simulink model "AFC1_F_trainrp_15_15_15_15_controller_ep_1000_Nor_20250519"  (R2021a)
settings: Solver=VariableStepAuto  StartTime=0.0  StopTime=10.0  RelTol=1e-3
libraries: neural x66
(part 3 of 3)

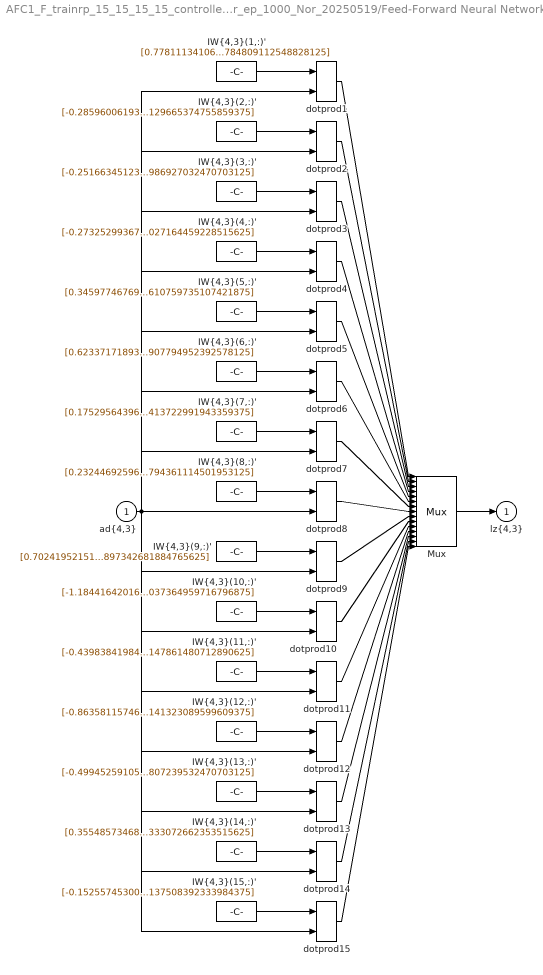
== system AFC1_F_trainrp_15_15_15_15_controller_ep_1000_Nor_20250519/Feed-Forward Neural Network/Layer 4/LW{4,3} ==
  "ad{4,3}" : Inport  PortDimensions=15
      mask Display: e = 0.06;c1 = [120 230 180]/255;c2 = ([120 230 180]+0)/(256+128);c3 = ([120 230 180]+128)/(256+128);patch([0 1 1 0],[0 0 1 1],c1);patch([0 1 1 1-e 1-e 0+e],[0 0 1 1-e 0+e 0+e],c2);patch([0 0 1 1-e 0+e 0+e],[0 1 1 1-e 1-e 0+e],c3);plot([0 1 1 0 0],[0 0 1 1 0]);
  "IW{4,3}(1,:)'" : Constant  Value=[0.7781113410617930270518627366982400417327880859375;0.62119814230305447910751581730437465012073516845703125;0.1907724978485869360422810814270633272826671600341796875;-0.29778807948838326158380596098140813410282135009765625;0.4547541881890297954527113688527606427669525146484375;-0.1544121990389732690385216073991614393889904022216796875;0.2058191613042310852410565757963922806084156036376953125;-0.404746974372004630904342548092245124280452728271484375;-0.839846360988684370596502049011178314685821533203125;0.579024458134550723542588457348756492137908935546875;1.092536353292825612726346662384457886219024658203125;0.862223254974441299935961069422774016857147216796875;0.447329224035958816774183333109249360859394073486328125;0.0023547517412946007697716055417913594283163547515869140625;0.460295474695853912283638464941759593784809112548828125]
      mask Display: e = 0.06;c1 = [120 150 230]/255;c2 = ([120 150 230]+0)/383;c3 = ([120 150 230]+128)/383;patch([0 1 1 0],[0 0 1 1],c1);patch([0 1 1 1-e 1-e 0+e],[0 0 1 1-e 0+e 0+e],c2);patch([0 0 1 1-e 0+e 0+e],[0 1 1 1-e 1-e 0+e],c3);plot([0 1 1 0 0],[0 0 1 1 0]);disp('weights');
  "IW{4,3}(10,:)'" : Constant  Value=[-1.18441642016053538810638201539404690265655517578125;0.71993919466000033668962032606941647827625274658203125;-0.73299228067737554059846161180757917463779449462890625;-1.0882850578337208702350835665129125118255615234375;-0.81389689755870031628859351258142851293087005615234375;0.80767521116610485609754732649889774620532989501953125;-0.255363153886374261158920262460014782845973968505859375;0.81081009055198982604650836947257630527019500732421875;-0.1617382409373282758924261770516750402748584747314453125;-1.1032546147443571538104833962279371917247772216796875;-0.26763008853710334999931319543975405395030975341796875;-0.5958498069031368249426350303110666573047637939453125;0.392774132323866098648323941233684308826923370361328125;-0.94132002652209190163290486452751792967319488525390625;-0.764998725995059469795478435116820037364959716796875]
      mask Display: e = 0.06;c1 = [120 150 230]/255;c2 = ([120 150 230]+0)/383;c3 = ([120 150 230]+128)/383;patch([0 1 1 0],[0 0 1 1],c1);patch([0 1 1 1-e 1-e 0+e],[0 0 1 1-e 0+e 0+e],c2);patch([0 0 1 1-e 0+e 0+e],[0 1 1 1-e 1-e 0+e],c3);plot([0 1 1 0 0],[0 0 1 1 0]);disp('weights');
  "IW{4,3}(11,:)'" : Constant  Value=[-0.43983841984739246999680517546948976814746856689453125;-0.217478877984103424747530652894056402146816253662109375;0.272952199327606448431282615274540148675441741943359375;-0.21779301126090844231697474242537282407283782958984375;-0.45534616982127251727519023916102014482021331787109375;1.2993100395773005129029797899420373141765594482421875;-0.4494260973686199367449489727732725441455841064453125;0.357711341633862922595454847396467812359333038330078125;-0.05326556157685528869460966916449251584708690643310546875;-0.72116789147178561591999823576770722866058349609375;2.368876520452326328580738845630548894405364990234375;-0.0922130686389561748939058816176839172840118408203125;-0.2799379158284567292724887010990642011165618896484375;-0.6096502573568012284255246413522399961948394775390625;0.5506923237256984293708228506147861480712890625]
      mask Display: e = 0.06;c1 = [120 150 230]/255;c2 = ([120 150 230]+0)/383;c3 = ([120 150 230]+128)/383;patch([0 1 1 0],[0 0 1 1],c1);patch([0 1 1 1-e 1-e 0+e],[0 0 1 1-e 0+e 0+e],c2);patch([0 0 1 1-e 0+e 0+e],[0 1 1 1-e 1-e 0+e],c3);plot([0 1 1 0 0],[0 0 1 1 0]);disp('weights');
  "IW{4,3}(12,:)'" : Constant  Value=[-0.86358115746454167105383703528787009418010711669921875;-0.12175056878691854767016167215842870064079761505126953125;-1.235565139600912853978798011667095124721527099609375;0.54022067020387087854516039442387409508228302001953125;0.260195066414997289161448179584112949669361114501953125;0.1290031436642831152994403964839875698089599609375;0.128307481278283452841293410529033280909061431884765625;-1.004774450547227804264593942207284271717071533203125;0.22686108419182193784990886342711746692657470703125;0.28467402097110283687442233713227324187755584716796875;4.31289008479221624980937122018076479434967041015625;-0.1441781603596583583026813357719220221042633056640625;-0.09857525629320285087686670522089116275310516357421875;0.51216925494200860047300238875322975218296051025390625;-0.24044180716196483782454151878482662141323089599609375]
      mask Display: e = 0.06;c1 = [120 150 230]/255;c2 = ([120 150 230]+0)/383;c3 = ([120 150 230]+128)/383;patch([0 1 1 0],[0 0 1 1],c1);patch([0 1 1 1-e 1-e 0+e],[0 0 1 1-e 0+e 0+e],c2);patch([0 0 1 1-e 0+e 0+e],[0 1 1 1-e 1-e 0+e],c3);plot([0 1 1 0 0],[0 0 1 1 0]);disp('weights');
  "IW{4,3}(13,:)'" : Constant  Value=[-0.49945259105140060729155493390862829983234405517578125;0.184426822089112152358580942745902575552463531494140625;-0.2031486968824770256158984693684033118188381195068359375;0.154916364295855479848995628344709984958171844482421875;0.9878538278918593817934379330836236476898193359375;0.0381209561733983626208299710924620740115642547607421875;-0.128199236742127464783180812446516938507556915283203125;0.3915529342565715609225662774406373500823974609375;0.96483039652991831047756932093761861324310302734375;0.78770085159116487449892929362249560654163360595703125;0.72610873909690687444395962302223779261112213134765625;0.93210549922399810185424939845688641071319580078125;-0.2202202028156553803572847982650273479521274566650390625;0.3195681221012935946390598473954014480113983154296875;0.7754075786498131339641304293763823807239532470703125]
      mask Display: e = 0.06;c1 = [120 150 230]/255;c2 = ([120 150 230]+0)/383;c3 = ([120 150 230]+128)/383;patch([0 1 1 0],[0 0 1 1],c1);patch([0 1 1 1-e 1-e 0+e],[0 0 1 1-e 0+e 0+e],c2);patch([0 0 1 1-e 0+e 0+e],[0 1 1 1-e 1-e 0+e],c3);plot([0 1 1 0 0],[0 0 1 1 0]);disp('weights');
  "IW{4,3}(14,:)'" : Constant  Value=[0.3554857346802153816867075875052250921726226806640625;-0.5248169129380049202637792404857464134693145751953125;0.683605962274300704706320175318978726863861083984375;-0.38434582116407411955805173420230858027935028076171875;0.58802983983653034361083200565190054476261138916015625;-0.646484905904349371752459774143062531948089599609375;0.4873657136989908433832852097111754119396209716796875;-0.1649823515269743523514733851698110811412334442138671875;0.356497028654995773422342608682811260223388671875;0.8647425210295389685910549815162084996700286865234375;0.53845365213304197116173099857405759394168853759765625;0.240110108266947452904105375637300312519073486328125;0.54410928450107098885979439728544093668460845947265625;0.53165142303777546128884523568558506667613983154296875;0.11257004837542540498507293023067177273333072662353515625]
      mask Display: e = 0.06;c1 = [120 150 230]/255;c2 = ([120 150 230]+0)/383;c3 = ([120 150 230]+128)/383;patch([0 1 1 0],[0 0 1 1],c1);patch([0 1 1 1-e 1-e 0+e],[0 0 1 1-e 0+e 0+e],c2);patch([0 0 1 1-e 0+e 0+e],[0 1 1 1-e 1-e 0+e],c3);plot([0 1 1 0 0],[0 0 1 1 0]);disp('weights');
  "IW{4,3}(15,:)'" : Constant  Value=[-0.15255745300140655107412612778716720640659332275390625;0.192276935283892225214685822720639407634735107421875;0.365743272093718096993342214773292653262615203857421875;0.6642693326831243805230542420758865773677825927734375;-0.215703456330019249787000035212258808314800262451171875;0.51382696907147706877339032871532253921031951904296875;0.398357784627120292686441871410352177917957305908203125;-0.309159641667459961222874653685721568763256072998046875;-0.650752509275324797499706619419157505035400390625;-0.454387145055632990509053570349351502954959869384765625;0.702470078125212893382922629825770854949951171875;0.3907799038360071364195391652174293994903564453125;0.21374221137187865426909638699726201593875885009765625;-1.028661893935131299571139606996439397335052490234375;-0.11374116937851606878862043004119186662137508392333984375]
      mask Display: e = 0.06;c1 = [120 150 230]/255;c2 = ([120 150 230]+0)/383;c3 = ([120 150 230]+128)/383;patch([0 1 1 0],[0 0 1 1],c1);patch([0 1 1 1-e 1-e 0+e],[0 0 1 1-e 0+e 0+e],c2);patch([0 0 1 1-e 0+e 0+e],[0 1 1 1-e 1-e 0+e],c3);plot([0 1 1 0 0],[0 0 1 1 0]);disp('weights');
  "IW{4,3}(2,:)'" : Constant  Value=[-0.285960061930889020143098377957358025014400482177734375;0.08086592897482065833703046564551186747848987579345703125;0.209619332545560921321481373524875380098819732666015625;0.601640573903069242334140653838403522968292236328125;0.61417095990891035217629223552648909389972686767578125;-0.249905092514466076192292121049831621348857879638671875;-0.5886553210720730788807486533187329769134521484375;-0.08819411407162684735094870802640798501670360565185546875;0.54536337903716447517155074820038862526416778564453125;-0.81532331654258360931208926558610983192920684814453125;0.1070831469910651367882792328600771725177764892578125;-0.61843070398175559176934257266111671924591064453125;-0.30620961942477276096497007529251277446746826171875;0.303505148267826874164398986977175809442996978759765625;0.000422648562204752664683837792836129665374755859375]
      mask Display: e = 0.06;c1 = [120 150 230]/255;c2 = ([120 150 230]+0)/383;c3 = ([120 150 230]+128)/383;patch([0 1 1 0],[0 0 1 1],c1);patch([0 1 1 1-e 1-e 0+e],[0 0 1 1-e 0+e 0+e],c2);patch([0 0 1 1-e 0+e 0+e],[0 1 1 1-e 1-e 0+e],c3);plot([0 1 1 0 0],[0 0 1 1 0]);disp('weights');
  "IW{4,3}(3,:)'" : Constant  Value=[-0.251663451232154555814446439399034716188907623291015625;-0.90063132922669997260101126812514849007129669189453125;-0.5369097640000288773620695792487822473049163818359375;0.60719789471583462958648169660591520369052886962890625;-0.389331520200921044061459497243049554526805877685546875;1.74669172230102542897611783700995147228240966796875;0.58370198101816173075206961584626697003841400146484375;0.3476103853449876712744526230380870401859283447265625;-0.392289122738981976823424702160991728305816650390625;-0.85377902191131782583255471763550303876399993896484375;-0.24619643273685964945940440884442068636417388916015625;-0.482835497162455329345220889081247150897979736328125;0.17398084105062039395050987877766601741313934326171875;0.86714425514428927765919752346235327422618865966796875;-2.27164249781733662558735886705107986927032470703125]
      mask Display: e = 0.06;c1 = [120 150 230]/255;c2 = ([120 150 230]+0)/383;c3 = ([120 150 230]+128)/383;patch([0 1 1 0],[0 0 1 1],c1);patch([0 1 1 1-e 1-e 0+e],[0 0 1 1-e 0+e 0+e],c2);patch([0 0 1 1-e 0+e 0+e],[0 1 1 1-e 1-e 0+e],c3);plot([0 1 1 0 0],[0 0 1 1 0]);disp('weights');
  "IW{4,3}(4,:)'" : Constant  Value=[-0.2732529936785204061067133807227946817874908447265625;0.88748914037818427136272703137365169823169708251953125;-0.68055072784371095639954774014768190681934356689453125;0.125053153635659219933273789138183929026126861572265625;0.2283691504369806668517384196093189530074596405029296875;1.0179494024616639880065349643700756132602691650390625;0.455171078746453849905861943625495769083499908447265625;0.71073800219987537385435416581458412110805511474609375;-0.4655437715307171320233692313195206224918365478515625;-0.9015058953706809319328385754488408565521240234375;-0.3386358680194658798967566326609812676906585693359375;0.7957313696805983216364666077424772083759307861328125;0.043389264024203788583378127441392280161380767822265625;0.61046519646348162968507722325739450752735137939453125;0.073231450808178222278144176016212441027164459228515625]
      mask Display: e = 0.06;c1 = [120 150 230]/255;c2 = ([120 150 230]+0)/383;c3 = ([120 150 230]+128)/383;patch([0 1 1 0],[0 0 1 1],c1);patch([0 1 1 1-e 1-e 0+e],[0 0 1 1-e 0+e 0+e],c2);patch([0 0 1 1-e 0+e 0+e],[0 1 1 1-e 1-e 0+e],c3);plot([0 1 1 0 0],[0 0 1 1 0]);disp('weights');
  "IW{4,3}(5,:)'" : Constant  Value=[0.345977467695158524829679436152218841016292572021484375;0.55874418470221420829346925529534928500652313232421875;0.281540849166205642273297371502849273383617401123046875;0.348033471447639353169023479495081119239330291748046875;0.6848204049687172112470534557360224425792694091796875;1.3071885017548259266817467505461536347866058349609375;0.79997261480059600469161296132369898259639739990234375;0.1772593793514647686482277322284062393009662628173828125;-0.37757355775344103587798372245742939412593841552734375;-0.9290081605080360294124375286628492176532745361328125;-0.72678510581043986871208062439109198749065399169921875;0.1867237207722178826685421881848014891147613525390625;-0.6170095617719109082344175476464442908763885498046875;0.24489837888735965787390114201116375625133514404296875;0.0848989138507549589984790827656979672610759735107421875]
      mask Display: e = 0.06;c1 = [120 150 230]/255;c2 = ([120 150 230]+0)/383;c3 = ([120 150 230]+128)/383;patch([0 1 1 0],[0 0 1 1],c1);patch([0 1 1 1-e 1-e 0+e],[0 0 1 1-e 0+e 0+e],c2);patch([0 0 1 1-e 0+e 0+e],[0 1 1 1-e 1-e 0+e],c3);plot([0 1 1 0 0],[0 0 1 1 0]);disp('weights');
  "IW{4,3}(6,:)'" : Constant  Value=[0.62337171893468978911556632738211192190647125244140625;-0.4281062871592735685766228925785981118679046630859375;1.76120848003445029661406806553713977336883544921875;0.58994442178758477179911778875975869596004486083984375;0.88055284261421051805740489726304076611995697021484375;1.544483268331445113830113768926821649074554443359375;-0.4300995639503575329598561438615433871746063232421875;0.1494743217128160495121846906840801239013671875;-0.24861571998082343526448312331922352313995361328125;-0.2988629653361092319840963682509027421474456787109375;-3.00849394685011706229715855442918837070465087890625;0.0076801636936958406209896565997041761875152587890625;0.1241120911235495949398455195478163659572601318359375;-1.4993528570491803098008176675648428499698638916015625;-5.4762503181029433818594043259508907794952392578125]
      mask Display: e = 0.06;c1 = [120 150 230]/255;c2 = ([120 150 230]+0)/383;c3 = ([120 150 230]+128)/383;patch([0 1 1 0],[0 0 1 1],c1);patch([0 1 1 1-e 1-e 0+e],[0 0 1 1-e 0+e 0+e],c2);patch([0 0 1 1-e 0+e 0+e],[0 1 1 1-e 1-e 0+e],c3);plot([0 1 1 0 0],[0 0 1 1 0]);disp('weights');
  "IW{4,3}(7,:)'" : Constant  Value=[0.1752956439626247864271846310657565481960773468017578125;0.150326465682723731109859954813146032392978668212890625;0.3548175390778631754784555596415884792804718017578125;-0.1728174639016286651127529694349505007266998291015625;0.370798773362751188376051914019626565277576446533203125;-0.04971012500731140926202300533986999653279781341552734375;0.353451972904515410167647360140108503401279449462890625;-0.305915658154417346992204329580999910831451416015625;0.181307586165917855591800389447598718106746673583984375;-0.30983706229363694450995581064489670097827911376953125;0.59485331607430225187016503696213476359844207763671875;0.225619177671118276151673853746615350246429443359375;0.396606578216912419865280980957322753965854644775390625;0.1834798767971686783706530832205316983163356781005859375;-0.2429693816001007034000025441855541430413722991943359375]
      mask Display: e = 0.06;c1 = [120 150 230]/255;c2 = ([120 150 230]+0)/383;c3 = ([120 150 230]+128)/383;patch([0 1 1 0],[0 0 1 1],c1);patch([0 1 1 1-e 1-e 0+e],[0 0 1 1-e 0+e 0+e],c2);patch([0 0 1 1-e 0+e 0+e],[0 1 1 1-e 1-e 0+e],c3);plot([0 1 1 0 0],[0 0 1 1 0]);disp('weights');
  "IW{4,3}(8,:)'" : Constant  Value=[0.23244692596808180784506703275837935507297515869140625;1.039552473941219634667731952504254877567291259765625;0.59559164168821931983899276019656099379062652587890625;0.526773649188713388724636388360522687435150146484375;-0.58644708412978996392439512419514358043670654296875;-0.436625604723841542753604016979807056486606597900390625;0.36355980883610150566909169356222264468669891357421875;-0.017150798296506064577471306620282121002674102783203125;0.053840308531953484649790198091068305075168609619140625;-0.9766380177393207961955567952827550470829010009765625;0.705478431065432065594222876825369894504547119140625;0.6388444844637517494589928901405073702335357666015625;-0.217088928579525164419550264938152395188808441162109375;0.251809460810672847141944430404691956937313079833984375;-0.8880476852244190144602953296271152794361114501953125]
      mask Display: e = 0.06;c1 = [120 150 230]/255;c2 = ([120 150 230]+0)/383;c3 = ([120 150 230]+128)/383;patch([0 1 1 0],[0 0 1 1],c1);patch([0 1 1 1-e 1-e 0+e],[0 0 1 1-e 0+e 0+e],c2);patch([0 0 1 1-e 0+e 0+e],[0 1 1 1-e 1-e 0+e],c3);plot([0 1 1 0 0],[0 0 1 1 0]);disp('weights');
  "IW{4,3}(9,:)'" : Constant  Value=[0.7024195215143633763688058024854399263858795166015625;0.36835613425324298386698274043737910687923431396484375;0.1616770468534722560161043247717316262423992156982421875;0.1514457268262039135731100714110652916133403778076171875;0.273830959485176161916086812198045663535594940185546875;1.3094823153233836610098705932614393532276153564453125;-0.80337001220094828024542721323086880147457122802734375;0.38559116646626900859473607852123677730560302734375;-0.296555542751998135742041995399631559848785400390625;-0.0038908790515449933992975228846944446559064090251922607421875;-0.928396868794197249741273481049574911594390869140625;0.063778338985851501519164230558089911937713623046875;0.66554084135262814303501954782404936850070953369140625;-0.26046794064293699033640905327047221362590789794921875;-0.8080524622324978256671101917163468897342681884765625]
      mask Display: e = 0.06;c1 = [120 150 230]/255;c2 = ([120 150 230]+0)/383;c3 = ([120 150 230]+128)/383;patch([0 1 1 0],[0 0 1 1],c1);patch([0 1 1 1-e 1-e 0+e],[0 0 1 1-e 0+e 0+e],c2);patch([0 0 1 1-e 0+e 0+e],[0 1 1 1-e 1-e 0+e],c3);plot([0 1 1 0 0],[0 0 1 1 0]);disp('weights');
  Mux : Mux  Inputs=15
      mask Display: e = 0.06;c1 = [120 150 230]/255;c2 = ([120 150 230]+0)/383;c3 = ([120 150 230]+128)/383;patch([0 1 1 0],[0 0 1 1],c1);patch([0 1 1 1-e 1-e 0+e],[0 0 1 1-e 0+e 0+e],c2);patch([0 0 1 1-e 0+e 0+e],[0 1 1 1-e 1-e 0+e],c3);plot([0 1 1 0 0],[0 0 1 1 0]);disp('Mux');
  dotprod{1..15} (15 alike) : neural/Weight Functions/dotprod
  "lz{4,3}" : Outport
      mask Display: e = 0.06;c1 = [120 230 180]/255;c2 = ([120 230 180]+0)/(256+128);c3 = ([120 230 180]+128)/(256+128);patch([0 1 1 0],[0 0 1 1],c1);patch([0 1 1 1-e 1-e 0+e],[0 0 1 1-e 0+e 0+e],c2);patch([0 0 1 1-e 0+e 0+e],[0 1 1 1-e 1-e 0+e],c3);plot([0 1 1 0 0],[0 0 1 1 0]);
  wires:
  "IW{4,3}(1,:)'"/1 -> dotprod1/1
  "ad{4,3}"/1 -> dotprod1/2, dotprod2/2, dotprod3/2, dotprod4/2, dotprod5/2, dotprod6/2, dotprod7/2, dotprod8/2, dotprod9/2, dotprod10/2, dotprod11/2, dotprod12/2, dotprod13/2, dotprod14/2, dotprod15/2
  dotprod1/1 -> Mux/1
  "IW{4,3}(2,:)'"/1 -> dotprod2/1
  dotprod2/1 -> Mux/2
  "IW{4,3}(3,:)'"/1 -> dotprod3/1
  dotprod3/1 -> Mux/3
  "IW{4,3}(4,:)'"/1 -> dotprod4/1
  dotprod4/1 -> Mux/4
  "IW{4,3}(5,:)'"/1 -> dotprod5/1
  dotprod5/1 -> Mux/5
  "IW{4,3}(6,:)'"/1 -> dotprod6/1
  dotprod6/1 -> Mux/6
  "IW{4,3}(7,:)'"/1 -> dotprod7/1
  dotprod7/1 -> Mux/7
  "IW{4,3}(8,:)'"/1 -> dotprod8/1
  dotprod8/1 -> Mux/8
  "IW{4,3}(9,:)'"/1 -> dotprod9/1
  dotprod9/1 -> Mux/9
  "IW{4,3}(10,:)'"/1 -> dotprod10/1
  dotprod10/1 -> Mux/10
  "IW{4,3}(11,:)'"/1 -> dotprod11/1
  dotprod11/1 -> Mux/11
  "IW{4,3}(12,:)'"/1 -> dotprod12/1
  dotprod12/1 -> Mux/12
  "IW{4,3}(13,:)'"/1 -> dotprod13/1
  dotprod13/1 -> Mux/13
  "IW{4,3}(14,:)'"/1 -> dotprod14/1
  dotprod14/1 -> Mux/14
  "IW{4,3}(15,:)'"/1 -> dotprod15/1
  dotprod15/1 -> Mux/15
  Mux/1 -> "lz{4,3}"/1

== system AFC1_F_trainrp_15_15_15_15_controller_ep_1000_Nor_20250519/Feed-Forward Neural Network/Layer 5/Delays 1 ==
  "p{5}" : Inport  PortDimensions=15
      mask Display: e = 0.06;c1 = [120 230 180]/255;c2 = ([120 230 180]+0)/(256+128);c3 = ([120 230 180]+128)/(256+128);patch([0 1 1 0],[0 0 1 1],c1);patch([0 1 1 1-e 1-e 0+e],[0 0 1 1-e 0+e 0+e],c2);patch([0 0 1 1-e 0+e 0+e],[0 1 1 1-e 1-e 0+e],c3);plot([0 1 1 0 0],[0 0 1 1 0]);
  mux : Mux  Inputs=1
      mask Display: e = 0.06;c1 = [120 150 230]/255;c2 = ([120 150 230]+0)/383;c3 = ([120 150 230]+128)/383;patch([0 1 1 0],[0 0 1 1],c1);patch([0 1 1 1-e 1-e 0+e],[0 0 1 1-e 0+e 0+e],c2);patch([0 0 1 1-e 0+e 0+e],[0 1 1 1-e 1-e 0+e],c3);plot([0 1 1 0 0],[0 0 1 1 0]);disp('Mux')
  "pd{5,4}" : Outport
      mask Display: e = 0.06;c1 = [120 230 180]/255;c2 = ([120 230 180]+0)/(256+128);c3 = ([120 230 180]+128)/(256+128);patch([0 1 1 0],[0 0 1 1],c1);patch([0 1 1 1-e 1-e 0+e],[0 0 1 1-e 0+e 0+e],c2);patch([0 0 1 1-e 0+e 0+e],[0 1 1 1-e 1-e 0+e],c3);plot([0 1 1 0 0],[0 0 1 1 0]);
  wires:
  "p{5}"/1 -> mux/1
  mux/1 -> "pd{5,4}"/1

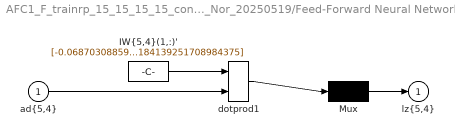
== system AFC1_F_trainrp_15_15_15_15_controller_ep_1000_Nor_20250519/Feed-Forward Neural Network/Layer 5/LW{5,4} ==
  "ad{5,4}" : Inport  PortDimensions=15
      mask Display: e = 0.06;c1 = [120 230 180]/255;c2 = ([120 230 180]+0)/(256+128);c3 = ([120 230 180]+128)/(256+128);patch([0 1 1 0],[0 0 1 1],c1);patch([0 1 1 1-e 1-e 0+e],[0 0 1 1-e 0+e 0+e],c2);patch([0 0 1 1-e 0+e 0+e],[0 1 1 1-e 1-e 0+e],c3);plot([0 1 1 0 0],[0 0 1 1 0]);
  "IW{5,4}(1,:)'" : Constant  Value=[-0.06870308859968256298689226468923152424395084381103515625;0.08721825140375678853121854672281187959015369415283203125;0.173572582455316426486291447872645221650600433349609375;-0.87607470177891222373744994911248795688152313232421875;0.232223904345521814374109226264408789575099945068359375;-0.060384389916776741447090870451575028710067272186279296875;-0.728766761237137128404128816328011453151702880859375;0.87711572866368481271592827397398650646209716796875;0.09614604588366688908696033877276931889355182647705078125;-0.0263306384783197622301287310619954951107501983642578125;-0.08828216693490435751368039518638397566974163055419921875;0.286897328779983584734480928091215901076793670654296875;-0.15339478556095909045353664623689837753772735595703125;0.59499409118017398956368424478569068014621734619140625;0.0022470049486926178816670329752014367841184139251708984375]
      mask Display: e = 0.06;c1 = [120 150 230]/255;c2 = ([120 150 230]+0)/383;c3 = ([120 150 230]+128)/383;patch([0 1 1 0],[0 0 1 1],c1);patch([0 1 1 1-e 1-e 0+e],[0 0 1 1-e 0+e 0+e],c2);patch([0 0 1 1-e 0+e 0+e],[0 1 1 1-e 1-e 0+e],c3);plot([0 1 1 0 0],[0 0 1 1 0]);disp('weights');
  Mux : Mux  Inputs=1
      mask Display: e = 0.06;c1 = [120 150 230]/255;c2 = ([120 150 230]+0)/383;c3 = ([120 150 230]+128)/383;patch([0 1 1 0],[0 0 1 1],c1);patch([0 1 1 1-e 1-e 0+e],[0 0 1 1-e 0+e 0+e],c2);patch([0 0 1 1-e 0+e 0+e],[0 1 1 1-e 1-e 0+e],c3);plot([0 1 1 0 0],[0 0 1 1 0]);disp('Mux');
  dotprod1 : neural/Weight Functions/dotprod
  "lz{5,4}" : Outport
      mask Display: e = 0.06;c1 = [120 230 180]/255;c2 = ([120 230 180]+0)/(256+128);c3 = ([120 230 180]+128)/(256+128);patch([0 1 1 0],[0 0 1 1],c1);patch([0 1 1 1-e 1-e 0+e],[0 0 1 1-e 0+e 0+e],c2);patch([0 0 1 1-e 0+e 0+e],[0 1 1 1-e 1-e 0+e],c3);plot([0 1 1 0 0],[0 0 1 1 0]);
  wires:
  "IW{5,4}(1,:)'"/1 -> dotprod1/1
  "ad{5,4}"/1 -> dotprod1/2
  dotprod1/1 -> Mux/1
  Mux/1 -> "lz{5,4}"/1
